simulink model "mte484lab2partb"  (R2024a)
settings: Solver=VariableStepAuto  StartTime=0.0  StopTime=10.0  MaxStep=0.001  RelTol=1e-3
values from neighbouring files (symbols this model uses):
  A = 1.0    (= 1)    [mte484lab2asetup.m]
  Cden = [1 pc]    [mte484lab2asetup.m]
  Cnum = -k*[1 zc]    [mte484lab2asetup.m]
  freq = 0.5    [mte484lab2asetup.m]
  K1 = -1.883    [lab2a_data.mat]    (also in lab2b_data.mat; mte484lab2asetup.m)
  sat = 0.7    [mte484lab2asetup.m]
  tau = 0.0216    [lab2a_data.mat]    (also in lab2b_data.mat; mte484lab2asetup.m)
  Ts = 0.001    [lab2b_data.mat]    (also in mte484lab2asetup.m; mte484lab2partbsetup.m)
undefined symbols (not defined in the file or in its folder): Dden, Dnum
settings Model: Creator=christopherkoo  LastModifiedBy=christopherkoo

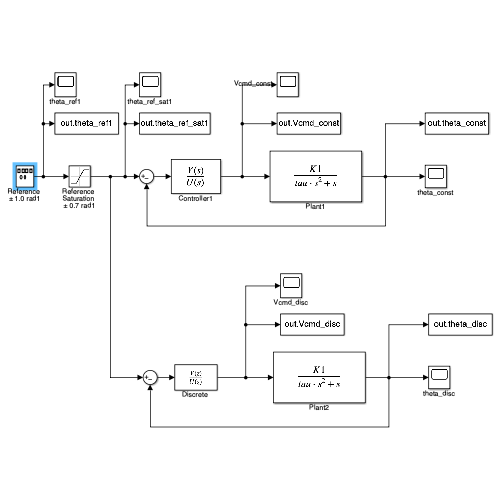
[thumbnail: Simulink's stored preview of the top-level diagram]
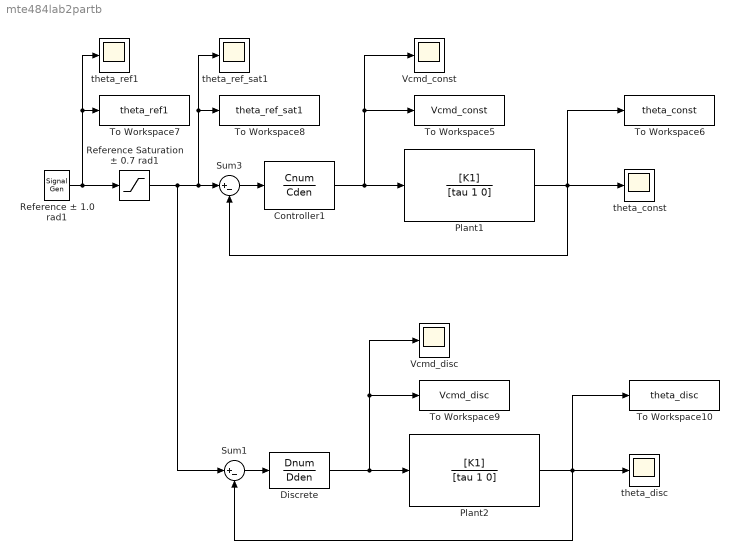
== system mte484lab2partb ==
  Controller1 : TransferFcn  Numerator=Cnum  Denominator=Cden
  "Discrete " : DiscreteTransferFcn  Numerator=Dnum  Denominator=Dden  SampleTime=Ts
  Plant1 : TransferFcn  Numerator=[K1]  Denominator=[tau 1 0]
  Plant2 : TransferFcn  Numerator=[K1]  Denominator=[tau 1 0]
  Reference Saturation ± 0.7 rad1 : Saturate  UpperLimit=sat  LowerLimit=-sat
  Reference ± 1.0 rad1 : SignalGenerator  WaveForm=square  Amplitude=A  Frequency=freq
  Sum1 : Sum  Inputs=|+-
  Sum3 : Sum  Inputs=|+-
  To Workspace10 : ToWorkspace  VariableName=theta_disc  SaveFormat=Timeseries  SampleTime=-1
  To Workspace5 : ToWorkspace  VariableName=Vcmd_const  SaveFormat=Timeseries  SampleTime=-1
  To Workspace6 : ToWorkspace  VariableName=theta_const  SaveFormat=Timeseries  SampleTime=-1
  To Workspace7 : ToWorkspace  VariableName=theta_ref1  SaveFormat=Timeseries  SampleTime=-1
  To Workspace8 : ToWorkspace  VariableName=theta_ref_sat1  SaveFormat=Timeseries  SampleTime=-1
  To Workspace9 : ToWorkspace  VariableName=Vcmd_disc  SaveFormat=Timeseries  SampleTime=-1
  Vcmd_const : Scope
  Vcmd_disc : Scope
  theta_const : Scope
  theta_disc : Scope
  theta_ref1 : Scope
  theta_ref_sat1 : Scope
  wires:
  Plant1/1 -> To Workspace6/1, theta_const/1, Sum3/2
  Reference Saturation ± 0.7 rad1/1 -> theta_ref_sat1/1, To Workspace8/1, Sum3/1, Sum1/1
  Reference ± 1.0 rad1/1 -> Reference Saturation ± 0.7 rad1/1, theta_ref1/1, To Workspace7/1
  Controller1/1 -> Plant1/1, Vcmd_const/1, To Workspace5/1
  Sum1/1 -> "Discrete "/1
  Sum3/1 -> Controller1/1
  Plant2/1 -> To Workspace10/1, theta_disc/1, Sum1/2
  "Discrete "/1 -> Plant2/1, Vcmd_disc/1, To Workspace9/1
